simulink model "Speed_control_of_wound_field_synchronous_motor_drive"  (R2024a)
settings: Solver=FixedStepDiscrete  StartTime=0.0  StopTime=1  FixedStep=Ts  RelTol=1e-3  EnableMultiTasking=on
PreLoadFcn:
  | SMDriveData;
undefined symbols (not defined in the file): Kt, Ts
libraries: nesl_utility x15, fl_lib x10, ee_lib x6, eeSmFieldOrientedControl x1, batteryecm_lib x1
CloseFcn:
  | try,close(h1_SMDrive),end
  | clear h1_SMDrive
  | 
  | clear simlog_SMDrive
  | clear logsout_SMDrive
Description:
  | Three-Phase Synchronous Machine Drive
settings Model: Creator=The MathWorks, Inc.  LastModifiedBy=haris
settings SolverCC: AlgebraicLoopSolver=TrustRegion  AutoInsertRateTranBlk=on  MaxZcPerStep=1
settings DataIOCC: MaxDataPoints=210000  ReturnWorkspaceOutputs=off  SignalLoggingName=logsout_SMDrive
settings OptimizationCC: ReuseModelBlockBuffer=off  LifeSpan=inf
settings DebuggingCC: UnconnectedInputMsg=warning  UnconnectedOutputMsg=warning  UnconnectedLineMsg=warning  SFUnexpectedBacktrackingDiag=warning  SFNoUnconditionalDefaultTransitionDiag=warning  SFExecutionAtInitializationDiag=none  ArithmeticOperatorsInVariantConditions=warning
settings ModelReferenceCC: EnableRefExpFcnMdlSchedulingChecks=on
settings SFSimCC: SimUseLocalCustomCode=off  CustomCodeUndefinedFunction=UseInterfaceOnly
settings RTWCC: RTWUseLocalCustomCode=off  GPUComputeCapability=3.5  DLArmComputeVersion=19.05
settings CodeAppCC: StateflowObjectComments=on
settings GRTTargetCC: TargetLangStandard=C89/C90 (ANSI)
settings ConfigComp: CovMetricSettings=dw  CovSaveCumulativeToWorkspaceVar=on  CovSaveSingleToWorkspaceVar=on  CovExternalEMLEnable=off
settings SimscapeCC: SimscapeLogType=all  SimscapeLogSimulationStatistics=on  SimscapeLogName=simlog_SMDrive  SimscapeLogDataHistory=210000

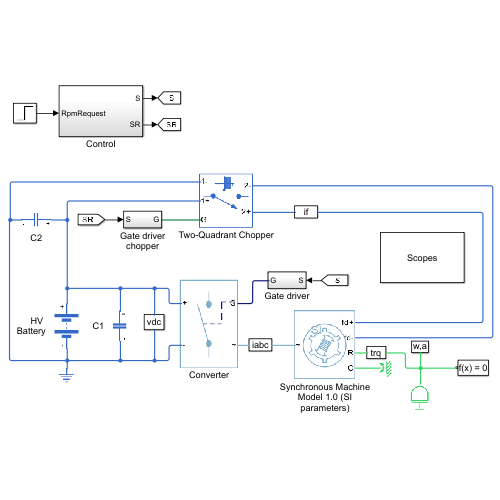
[thumbnail: Simulink's stored preview of the top-level diagram]
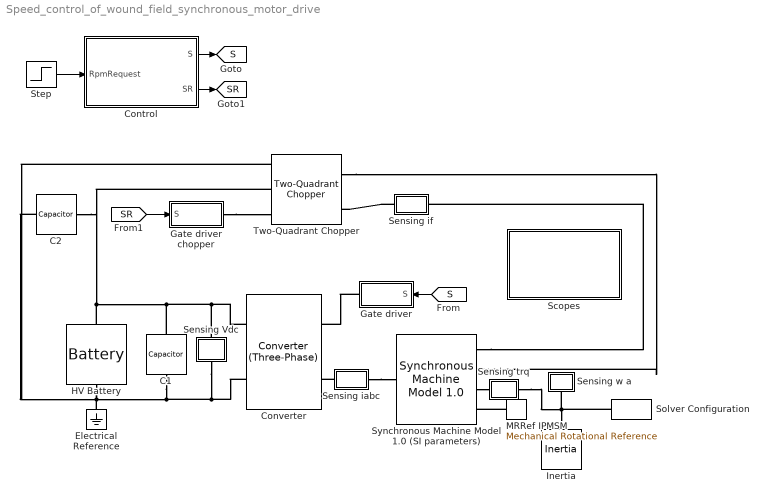
== system Speed_control_of_wound_field_synchronous_motor_drive ==
  C1 : fl_lib/Electrical/Electrical Elements/Capacitor  c=Cdc F  r=1e-6 Ohm  g=0 1/Ohm  i_specify=off  i_priority=None  i=0 A  i_nominal_specify=off  i_nominal_value=1  i_nominal_unit=A  v_specify=off  v_priority=None  v=0 V  v_nominal_specify=off  v_nominal_value=1  v_nominal_unit=V  vc_specify=on  vc_priority=None  vc=Vnom V  vc_nominal_specify=off  vc_nominal_value=1  vc_nominal_unit=V
  C2 : fl_lib/Electrical/Electrical Elements/Capacitor  c=Cdc F  r=1e-6 Ohm  g=0 1/Ohm  i_specify=off  i_priority=None  i=0 A  i_nominal_specify=off  i_nominal_value=1  i_nominal_unit=A  v_specify=off  v_priority=None  v=0 V  v_nominal_specify=off  v_nominal_value=1  v_nominal_unit=V  vc_specify=on  vc_priority=None  vc=Vnom V  vc_nominal_specify=off  vc_nominal_value=1  vc_nominal_unit=V
  Control : Subsystem
  Converter : ee_lib/Semiconductors & Converters/Converters/Converter (Three-Phase)  port_option=ee.enum.threePhasePort.composite  fidelity_option=ee.enum.converters.fidelity.detailed  device_type=2  K=0  Vf=0.8 V  Ron=0.001 Ohm  Rds=0.001 Ohm  Goff=1e-5 1/Ohm  Vgt=1 V  Vgt_off=-1 V  Ih=1 A  Vth=0.5 V  diode_param=2  diode_Vf=0.8 V  diode_Ron=0.001 Ohm  diode_Goff=1e-5 1/Ohm  diode_C=50 nF  diode_iRM=-235 A  diode_iF=300 A  diode_idot=-50 A/us  diode_trr_param=1  diode_trr_factor=3  diode_trr=15 us  diode_Qrr=1.5e+3 s*uA  snubber_type=0  Cs=1e-7 F  Rs=0.1 Ohm
  Electrical Reference : fl_lib/Electrical/Electrical Elements/Electrical Reference
  Gate driver : Subsystem
  Gate driver chopper : Subsystem
  HV Battery : batteryecm_lib/Battery  Vnom=Vnom V  prm_dir=1  R1_dis=2 Ohm  R1_ch=2 Ohm  R1=0.001 Ohm  prm_AH=1  AH=300 hr*A  V1=330 V  AH1=100 hr*A  prm_R2=1  R2=2000 Ohm  Tmeas=298.15 K  charge_measurement_port=simscape.enum.battery.enable.no  prm_dyn=1  Rp1=0.005 Ohm  tau1=30 s  Rp2=0.005 Ohm  tau2=30 s  Rp3=0.005 Ohm  tau3=30 s  Rp4=0.005 Ohm  tau4=30 s  Rp5=0.005 Ohm  tau5=30 s  prm_fade=1  N_fade=100  AH_fade=45 hr*A  R1_fade=2.02 Ohm  R1_ch_fade=2.02 Ohm  V1_fade=10.35 V  prm_age=1  prm_age_OCV=1  OCV_age=0.9  SOC_age=60  Tmeas_age=298.15 K  delta_time_age_vec=[0] d  temperature_age_vec=[273] K  OCV_scaling_age=2.2134e6  OCV_offset_age=1.632e6  temp_exp_age=0.515833569 V  t_exp_age=0.75  Vnom_T2=12 V  R1_T2=2.2 Ohm  R1_T2_dis=2.2 Ohm  R1_T2_ch=2.2 Ohm  V1_T2=11.4 V  R2_T2=2200 Ohm  Rp1_T2=0.005 Ohm  tau1_T2=30 s  Rp2_T2=0.005 Ohm  tau2_T2=30 s  Rp3_T2=0.005 Ohm  tau3_T2=30 s  Rp4_T2=0.005 Ohm  tau4_T2=30 s  Rp5_T2=0.005 Ohm  tau5_T2=30 s  Tmeas2=273.15 K  thermal_port=simscape.enum.thermaleffects.omit  thermal_mass=30000 J/K  i_specify=off  i_priority=None  i=0 A  i_nominal_specify=off  i_nominal_value=1  i_nominal_unit=A  v_specify=off  v_priority=None  v=0 V  v_nominal_specify=off  v_nominal_value=1  v_nominal_unit=V  charge_specify=on  charge_priority=High  charge=100 hr*A  charge_nominal_specify=off  charge_nominal_value=1  charge_nominal_unit=A*hr  num_cycles_specify=off  num_cycles_priority=High  num_cycles=0  num_cycles_nominal_specify=off  num_cycles_nominal_value=1  num_cycles_nominal_unit=1  temperature_specify=off  temperature_priority=High  temperature=298.15 K  temperature_nominal_specify=off  temperature_nominal_value=1  temperature_nominal_unit=K
  Inertia : fl_lib/Mechanical/Rotational Elements/Inertia  inertia=Jm kg*m^2  num_ports=foundation.enum.numPorts2.one  w_specify=on  w_priority=High  w=0 rpm  w_nominal_specify=off  w_nominal_value=1  w_nominal_unit=rad/s  t_specify=off  t_priority=High  t=0 N*m  t_nominal_specify=off  t_nominal_value=1  t_nominal_unit=N*m
  MRRef IPMSM : fl_lib/Mechanical/Rotational Elements/Mechanical Rotational Reference
  Scopes : Subsystem
      mask Display: disp(get_param(gcb,'Name'))
  Sensing Vdc : Subsystem
      mask Display: disp('vdc')
  Sensing trq : Subsystem
      mask Display: disp('trq')
  Sensing w a : Subsystem
      mask Display: disp('w,a')
  Sensing iabc : Subsystem
      mask Display: disp('iabc')
  Sensing if : Subsystem
      mask Display: disp('if')
  Solver Configuration : nesl_utility/Solver Configuration  PhysicalDomain=network_engine_domain  SubClassName=solver  LeftPortType=input  RightPortType=generic  Tones=[]  Harmonics=[]  SimulateNoise=off  Profile=off  UseLocalSampling=off  EnableSwitchedLinearOptims=on  FrequencyDomain=off  UseCCode=off  RelTol=0.001  AbsTol=1e-06  MinStep=1e-09  ToWorkspace=off  RevertToSquareIcSolve=off  NumHomotopyIterations=100  PhasorMode=off  PhasorModeNumHarmonics=1  ConsistencySolver=NEWTON_FTOL  IndexReductionMethod=DerivativeReplacement  DoDC=off  ResidualTolerance=1e-9  ConsistencyTolSource=GLOBAL  ConsistencyAbsTol=0.001  ConsistencyRelTol=0.001  ConsistencyTolFactor=0.001  UseLocalSolver=on  LocalSolverChoice=NE_BACKWARD_EULER_ADVANCER  ResolveIndetEquations=on  FunctionEvalNumThread=1  LocalSolverSampleTime=Ts  DoFixedCost=on  MaxNonlinIter=4  MaxModeIter=2  ComputeImpulses=off  ImpulseIterations=2  LinearAlgebra=auto  LinearAlgebraNumThread=0  EquationFormulation=NE_TIME_EF  DelaysMemoryBudget=1024  AutomaticFiltering=on  FilteringTimeConstant=0.001  PartitionStorageMethod=AS_NEEDED  PartitionMemoryBudget=1024  PartitionMethod=FAST  MultibodyUseLocalSolver=off  MultibodyLocalSolverChoice=ODE1  MultibodyLocalSolverSampleTime=0.001
  Step : Step  Time=0.1  After=1500  SampleTime=0
  Synchronous Machine Model 1.0 (SI parameters) : ee_lib/Electromechanical/Synchronous/Synchronous Machine Model 1.0  port_option=ee.enum.threePhasePort.composite  winding_type=ee.enum.electromech.statorconfiguration.wye  machine_param=ee.enum.pmsm.hybridparameterization.constant  nPolePairs=p  stator_param=1  Ld=Ld H  Lq=Lq H  idVec=[-200, 0, 200] A  iqVec=[-200, 0, 200] A  ifVec=[-20, 0, 20] A  LdMatrix=0.00015 * ones(3, 3, 3) H  LqMatrix=0.00021 * ones(3, 3, 3) H  LmfMatrix=0.007 * ones(3, 3, 3) H  LfVec=0.5 * ones(1, 3) H  L0=L0 H  Ls=0.00016 H  Lm=-0.00002 H  Ms=0.00002 H  Lf=Lf H  Lmf=Lmf H  Rs=Rs Ohm  Rf=Rf Ohm  zero_sequence=ee.enum.park.zerosequence.exclude  J=0 kg*m^2  lam=0 N*m/(rad/s)  axes_param=1  i_d_specify=off  i_d_priority=None  i_d=0 A  i_d_nominal_specify=off  i_d_nominal_value=1  i_d_nominal_unit=A  i_q_specify=off  i_q_priority=None  i_q=0 A  i_q_nominal_specify=off  i_q_nominal_value=1  i_q_nominal_unit=A  i_f_specify=off  i_f_priority=None  i_f=0 A  i_f_nominal_specify=off  i_f_nominal_value=1  i_f_nominal_unit=A  torque_specify=off  torque_priority=None  torque=0 N*m  torque_nominal_specify=off  torque_nominal_value=1  torque_nominal_unit=N*m  angular_velocity_specify=on  angular_velocity_priority=High  angular_velocity=0 rpm  angular_velocity_nominal_specify=off  angular_velocity_nominal_value=1  angular_velocity_nominal_unit=rpm  angular_position_diff_specify=on  angular_position_diff_priority=High  angular_position_diff=0 deg  angular_position_diff_nominal_specify=off  angular_position_diff_nominal_value=1  angular_position_diff_nominal_unit=deg  Tmeas=298.15 K  alpha=3.93e-3 1/K  stator_thermal_mass=100 J/K  rotor_thermal_mass=200 J/K  temperatureA_specify=off  temperatureA_priority=High  temperatureA=25 degC  temperatureA_nominal_specify=off  temperatureA_nominal_value=1  temperatureA_nominal_unit=degC  temperatureB_specify=off  temperatureB_priority=High  temperatureB=25 degC  temperatureB_nominal_specify=off  temperatureB_nominal_value=1  temperatureB_nominal_unit=degC  temperatureC_specify=off  temperatureC_priority=High  temperatureC=25 degC  temperatureC_nominal_specify=off  temperatureC_nominal_value=1  temperatureC_nominal_unit=degC  temperatureR_specify=off  temperatureR_priority=High  temperatureR=25 degC  temperatureR_nominal_specify=off  temperatureR_nominal_value=1  temperatureR_nominal_unit=degC
      settings: InternalSimscapePortConfiguration="{\"Bottom\":[],\"Left\":[{\"id\":\"N\",\"label\":\"~\",\"type\":\"foundation.electrical.three_phase\"}],\"Right\":[{\"id\":\"fd_p\",\"label\":\"fd+\",\"type\":\"foundation.electrical.electrical\"},{\"id\":\"fd_n\",\"label\":\"fd-\",\"type\":\"foundation.electrical.electrical\"},{\"id\":\"R\",\"label\":\"R\",\"type\":\"foundation.mechanical.rotational.rotational\"},{\"id\":\"C\",\"label\":\"C\",\"type\":\"foundation.mechanical.rotational.rotational\"}],\"Top\":[]}"
  Two-Quadrant Chopper : ee_lib/Semiconductors & Converters/Converters/Two-Quadrant Chopper  device_type=3  Vf=0.8 V  Ron=0.001 Ohm  Rds=0.001 Ohm  Goff=1e-5 1/Ohm  Vgt=1 V  Vgt_off=-1 V  Ih=1 A  Vth=0.5 V  K=0  diode_param=2  diode_Vf=0.8 V  diode_Ron=0.001 Ohm  diode_Goff=1e-5 1/Ohm  diode_C=50 nF  diode_iRM=-235 A  diode_iF=300 A  diode_idot=-50 A/us  diode_trr_param=1  diode_trr_factor=3  diode_trr=15 us  diode_Qrr=1500 s*uA  snubber_type=0  Cs=1e-7 F  Rs=0.1 Ohm
      settings: InternalSimscapePortConfiguration="{\"Bottom\":[],\"Left\":[{\"id\":\"G\",\"label\":\"G\",\"type\":\"foundation.electrical.four_phase\"},{\"id\":\"p1\",\"label\":\"1+\",\"type\":\"foundation.electrical.electrical\"},{\"id\":\"n1\",\"label\":\"1-\",\"type\":\"foundation.electrical.electrical\"}],\"Right\":[{\"id\":\"p2\",\"label\":\"2+\",\"type\":\"foundation.electrical.electrical\"},{\"id\":\"n2\",\"label\":\"2-\",\"type\":\"foundation.electrical.electrical\"}],\"Top\":[]}"
  tag scope: S=global, SR=global
  wires:
  [S] -> Gate driver/1(S)
  [SR] -> Gate driver chopper/1(S)
  Step/1 -> Control/1(RpmRequest)
  Control/1(S) -> [S]
  Control/2(SR) -> [SR]
  connections:
  Converter/RConn2 -- Sensing Vdc/RConn1 -- Two-Quadrant Chopper/LConn3 -- C2/RConn1 -- HV Battery/RConn1 -- Electrical Reference/LConn1 -- C1/RConn1
  Converter/RConn1 -- Sensing Vdc/LConn1 -- Two-Quadrant Chopper/LConn2 -- C2/LConn1 -- HV Battery/LConn1 -- C1/LConn1
  Gate driver/RConn1 -- Converter/LConn1
  Synchronous Machine Model 1.0 (SI parameters)/RConn1 -- Sensing if/RConn1
  Sensing iabc/LConn1 -- Converter/LConn2
  Sensing iabc/RConn1 -- Synchronous Machine Model 1.0 (SI parameters)/LConn1
  Solver Configuration/RConn1 -- Inertia/LConn1 -- Sensing trq/RConn1 -- Sensing w a/LConn1
  Synchronous Machine Model 1.0 (SI parameters)/RConn3 -- Sensing trq/LConn1
  MRRef IPMSM/LConn1 -- Synchronous Machine Model 1.0 (SI parameters)/RConn4
  Gate driver chopper/RConn1 -- Two-Quadrant Chopper/LConn1
  Two-Quadrant Chopper/RConn2 -- Synchronous Machine Model 1.0 (SI parameters)/RConn2
  Sensing if/LConn1 -- Two-Quadrant Chopper/RConn1

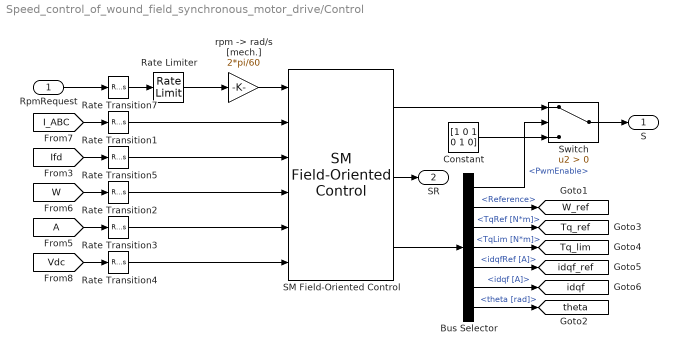
== system Speed_control_of_wound_field_synchronous_motor_drive/Control ==
  RpmRequest : Inport
  Bus Selector : BusSelector  OutputSignals=PwmEnable,Reference,TqRef [N*m],TqLim [N*m],idqfRef [A],idqf [A],theta [rad]
  Constant : Constant  Value=[1 0 1 0 1 0]
  From5 : From  TagVisibility=global
  Rate Limiter : RateLimiter  RisingSlewLimit=4000  FallingSlewLimit=-4000  SampleTimeMode=inherited
  Rate Transition{1..5,7} (6 alike) : RateTransition  OutPortSampleTime=Tsc
  SM Field-Oriented Control : eeSmFieldOrientedControl/SM Field-Oriented Control  CtrlMode=Velocity control  Vnom=Vnom  Pmax=Pmax  Tmax=Tmax  ifmax=ifmax  Vdc_on=100  p=p  Ts=Ts  Tsc=Tsc  CtrlType=PI control  Kp_w=Kp_omega  Ki_w=Ki_omega  Kv_w=1  Kaw_w=Kaw_omega  RefType=Zero d-axis control  rpmVec=[0, 3000]  TqVec=[-100, 0, 100]  VdcVec=[300, 350]  idMatrix=zeros(2,3,2)  iqMatrix=zeros(2,3,2)  ifMatrix=zeros(2,3,2)  Kt=Kt  AxisAlignment=Q-axis  Kp_id=Kp_id  Ki_id=Ki_id  Kaw_id=Kaw_id  Kp_iq=Kp_iq  Ki_iq=Ki_iq  Kaw_iq=Kaw_iq  Kp_if=Kp_if  Ki_if=Ki_if  Kaw_if=Kaw_if  AxisPrio=Q-axis  ActZC=on  ActFF=on  ParamTypeFF=Constant parameters  Ld=Ld  Lq=Lq  Lmf=Lmf  idVect=[-200, 200]  iqVect=[-200, 200]  ifVect=[0, 20]  LdMatrix=0.0002 * ones(2,2,2)  LqMatrix=0.0002 * ones(2,2,2)  LmfMatrix=0.007 * ones(2,2,2)  CPWMMode=SVM: space vector modulation  fsw=fsw  ChopperType=First and fourth quadrant chopper  fswe=fsw
      settings: SamplingMode=Natural
  Switch : Switch  Criteria=u2 > Threshold  SaturateOnIntegerOverflow=off  InputSameDT=off
  "rpm -> rad/s [mech.]" : Gain  Gain=2*pi/60
  S : Outport  VectorParamsAs1DForOutWhenUnconnected=off
  SR : Outport  Port=2  VectorParamsAs1DForOutWhenUnconnected=off
  tag scope: Tq_lim=global, Tq_ref=global, W_ref=global, idqf=global, idqf_ref=global, theta=global
  wires:
  [Ifd] -> Rate Transition5/1
  [W] -> Rate Transition2/1
  Rate Transition1/1 -> SM Field-Oriented Control/2
  [I_ABC] -> Rate Transition1/1
  From5/1 -> Rate Transition3/1
  RpmRequest/1 -> Rate Transition7/1
  [Vdc] -> Rate Transition4/1
  Rate Transition7/1 -> Rate Limiter/1
  "rpm -> rad/s [mech.]"/1 -> SM Field-Oriented Control/1
  SM Field-Oriented Control/2 -> SR/1
  SM Field-Oriented Control/3 -> Bus Selector/1
  Bus Selector/2 -> [W_ref]  "<Reference>"
  Bus Selector/7 -> [theta]  "<theta [rad]>"
  Bus Selector/3 -> [Tq_ref]  "<TqRef [N*m]>"
  Bus Selector/4 -> [Tq_lim]  "<TqLim [N*m]>"
  Bus Selector/5 -> [idqf_ref]  "<idqfRef [A]>"
  Bus Selector/6 -> [idqf]  "<idqf [A]>"
  Rate Limiter/1 -> "rpm -> rad/s [mech.]"/1
  Rate Transition5/1 -> SM Field-Oriented Control/3
  Rate Transition2/1 -> SM Field-Oriented Control/4
  Rate Transition3/1 -> SM Field-Oriented Control/5
  Rate Transition4/1 -> SM Field-Oriented Control/6
  SM Field-Oriented Control/1 -> Switch/1
  Switch/1 -> S/1
  Constant/1 -> Switch/3
  Bus Selector/1 -> Switch/2  "<PwmEnable>"

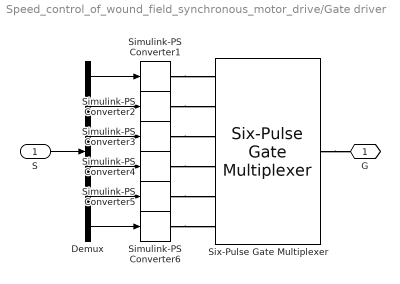
== system Speed_control_of_wound_field_synchronous_motor_drive/Gate driver ==
  S : Inport
  Demux : Demux  Outputs=6
  Simulink-PS Converter{1..6} (6 alike) : nesl_utility/Simulink-PS Converter  PhysicalDomain=network_engine_domain  SubClassName=ps_input  LeftPortType=input  RightPortType=output  PseudoPeriodic=off  Frequencies=[]  NoiseDistribution=none  NoiseParameters=[]  Unit=1  AffineConversion=off  FilteringAndDerivatives=zero  SimscapeFilterOrder=1  InputFilterTimeConstant=0.001  UdotUserProvided=1
  Six-Pulse Gate Multiplexer : ee_lib/Semiconductors & Converters/Converters/Six-Pulse Gate Multiplexer  port_option=ee.enum.controlport.ps
  G : PMIOPort  Side=Right
  wires:
  Demux/1 -> Simulink-PS Converter1/1
  S/1 -> Demux/1
  Demux/4 -> Simulink-PS Converter4/1
  Demux/2 -> Simulink-PS Converter2/1
  Demux/3 -> Simulink-PS Converter3/1
  Demux/5 -> Simulink-PS Converter5/1
  Demux/6 -> Simulink-PS Converter6/1
  connections:
  Six-Pulse Gate Multiplexer/RConn1 -- G/RConn1
  Simulink-PS Converter1/RConn1 -- Six-Pulse Gate Multiplexer/LConn1
  Simulink-PS Converter3/RConn1 -- Six-Pulse Gate Multiplexer/LConn3
  Simulink-PS Converter5/RConn1 -- Six-Pulse Gate Multiplexer/LConn5
  Simulink-PS Converter6/RConn1 -- Six-Pulse Gate Multiplexer/LConn6
  Simulink-PS Converter4/RConn1 -- Six-Pulse Gate Multiplexer/LConn4
  Simulink-PS Converter2/RConn1 -- Six-Pulse Gate Multiplexer/LConn2

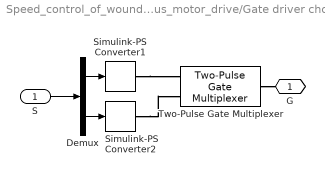
== system Speed_control_of_wound_field_synchronous_motor_drive/Gate driver chopper ==
  S : Inport
  Demux : Demux  Outputs=2
  Simulink-PS Converter1 : nesl_utility/Simulink-PS Converter  PhysicalDomain=network_engine_domain  SubClassName=ps_input  LeftPortType=input  RightPortType=output  PseudoPeriodic=off  Frequencies=[]  NoiseDistribution=none  NoiseParameters=[]  Unit=1  AffineConversion=off  FilteringAndDerivatives=zero  SimscapeFilterOrder=1  InputFilterTimeConstant=0.001  UdotUserProvided=1
  Simulink-PS Converter2 : nesl_utility/Simulink-PS Converter  PhysicalDomain=network_engine_domain  SubClassName=ps_input  LeftPortType=input  RightPortType=output  PseudoPeriodic=off  Frequencies=[]  NoiseDistribution=none  NoiseParameters=[]  Unit=1  AffineConversion=off  FilteringAndDerivatives=zero  SimscapeFilterOrder=1  InputFilterTimeConstant=0.001  UdotUserProvided=1
  Two-Pulse Gate Multiplexer : ee_lib/Semiconductors & Converters/Converters/Two-Pulse Gate Multiplexer  port_option=ee.enum.controlport.ps
      settings: InternalSimscapePortConfiguration="{\"Bottom\":[],\"Left\":[{\"id\":\"G1_ps\",\"label\":\"G1\",\"type\":\"input\"},{\"id\":\"G2_ps\",\"label\":\"G2\",\"type\":\"input\"}],\"Right\":[{\"id\":\"p\",\"label\":\"G\",\"type\":\"foundation.electrical.four_phase\"}],\"Top\":[]}"
  G : PMIOPort  Side=Right
  wires:
  Demux/1 -> Simulink-PS Converter1/1
  Demux/2 -> Simulink-PS Converter2/1
  S/1 -> Demux/1
  connections:
  Two-Pulse Gate Multiplexer/RConn1 -- G/RConn1
  Simulink-PS Converter1/RConn1 -- Two-Pulse Gate Multiplexer/LConn1
  Simulink-PS Converter2/RConn1 -- Two-Pulse Gate Multiplexer/LConn2

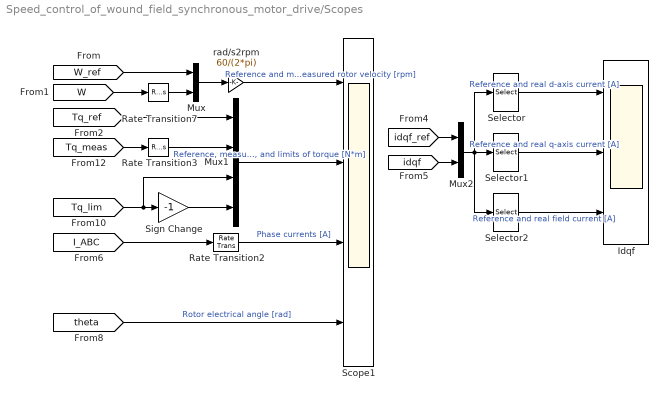
== system Speed_control_of_wound_field_synchronous_motor_drive/Scopes ==
  "Idqf " : Scope  NumInputPorts=3
  Mux : Mux  Inputs=2
  Mux1 : Mux
  Mux2 : Mux  Inputs=2
  Rate Transition2 : RateTransition
  Rate Transition3 : RateTransition
  Rate Transition7 : RateTransition
  Scope1 : Scope  NumInputPorts=4
  Selector : Selector  InputPortWidth=6  IndexOptions=Index vector (dialog)  Indices=[1 4]  OutputSizes=1
  Selector1 : Selector  InputPortWidth=6  IndexOptions=Index vector (dialog)  Indices=[2 5]  OutputSizes=1
  Selector2 : Selector  InputPortWidth=6  IndexOptions=Index vector (dialog)  Indices=[3 6]  OutputSizes=1
  Sign Change : Gain  Gain=-1
  rad/s2rpm : Gain  Gain=60/(2*pi)
  wires:
  Mux1/1 -> Scope1/2  "Reference, measured, and limits of torque [N*m]"
  Sign Change/1 -> Mux1/4
  Rate Transition3/1 -> Mux1/2
  [idqf] -> Mux2/2
  [W] -> Rate Transition7/1
  Selector/1 -> "Idqf "/1  "Reference and real d-axis current [A]"
  [I_ABC] -> Rate Transition2/1
  [idqf_ref] -> Mux2/1
  [theta] -> Scope1/4  "Rotor electrical angle [rad]"
  Mux2/1 -> Selector/1, Selector2/1, Selector1/1
  Selector1/1 -> "Idqf "/2  "Reference and real q-axis current [A]"
  [W_ref] -> Mux/1
  [Tq_meas] -> Rate Transition3/1
  Selector2/1 -> "Idqf "/3  "Reference and real field current [A]"
  [Tq_lim] -> Mux1/3, Sign Change/1
  Mux/1 -> rad/s2rpm/1
  Rate Transition2/1 -> Scope1/3  "Phase currents [A]"
  [Tq_ref] -> Mux1/1
  rad/s2rpm/1 -> Scope1/1  "Reference and measured rotor velocity [rpm]"
  Rate Transition7/1 -> Mux/2

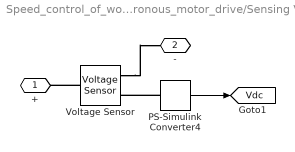
== system Speed_control_of_wound_field_synchronous_motor_drive/Sensing Vdc ==
  PS-Simulink Converter4 : nesl_utility/PS-Simulink Converter  PhysicalDomain=network_engine_domain  SubClassName=ps_output  LeftPortType=input  RightPortType=output  PseudoPeriodic=off  Frequencies=[]  VectorFormat=1-D array  Unit=V  AffineConversion=off
  Voltage Sensor : fl_lib/Electrical/Electrical Sensors/Voltage Sensor
  + : PMIOPort  Side=Left
  - : PMIOPort  Port=2  Side=Right
  tag scope: Vdc=global
  wires:
  PS-Simulink Converter4/1 -> [Vdc]
  connections:
  Voltage Sensor/LConn1 -- +/RConn1
  Voltage Sensor/RConn2 -- -/RConn1
  PS-Simulink Converter4/LConn1 -- Voltage Sensor/RConn1

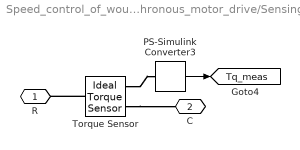
== system Speed_control_of_wound_field_synchronous_motor_drive/Sensing trq ==
  PS-Simulink Converter3 : nesl_utility/PS-Simulink Converter  PhysicalDomain=network_engine_domain  SubClassName=ps_output  LeftPortType=input  RightPortType=output  PseudoPeriodic=off  Frequencies=[]  VectorFormat=1-D array  Unit=N*m  AffineConversion=off
  Torque Sensor : fl_lib/Mechanical/Mechanical Sensors/Ideal Torque Sensor
  R : PMIOPort  Side=Left
  C : PMIOPort  Port=2  Side=Right
  tag scope: Tq_meas=global
  wires:
  PS-Simulink Converter3/1 -> [Tq_meas]
  connections:
  Torque Sensor/RConn1 -- C/RConn1
  Torque Sensor/RConn2 -- PS-Simulink Converter3/LConn1
  Torque Sensor/LConn1 -- R/RConn1

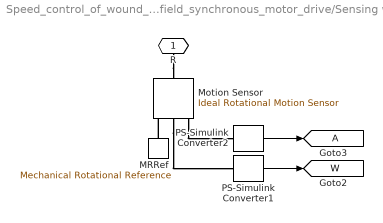
== system Speed_control_of_wound_field_synchronous_motor_drive/Sensing w a ==
  Goto3 : Goto  TagVisibility=global
  MRRef : fl_lib/Mechanical/Rotational Elements/Mechanical Rotational Reference
  Motion Sensor : fl_lib/Mechanical/Mechanical Sensors/Ideal Rotational Motion Sensor  reference=foundation.enum.MeasurementReference.difference  acceleration_port=false  velocity_port=true  position_port=true  wrap_angle=simscape.enum.onoff.off  offset=0 deg
  PS-Simulink Converter1 : nesl_utility/PS-Simulink Converter  PhysicalDomain=network_engine_domain  SubClassName=ps_output  LeftPortType=input  RightPortType=output  PseudoPeriodic=off  Frequencies=[]  VectorFormat=1-D array  Unit=rad/s  AffineConversion=off
  PS-Simulink Converter2 : nesl_utility/PS-Simulink Converter  PhysicalDomain=network_engine_domain  SubClassName=ps_output  LeftPortType=input  RightPortType=output  PseudoPeriodic=off  Frequencies=[]  VectorFormat=1-D array  Unit=rad  AffineConversion=off
  R : PMIOPort  Side=Left
  tag scope: W=global
  wires:
  PS-Simulink Converter1/1 -> [W]
  PS-Simulink Converter2/1 -> Goto3/1
  connections:
  R/RConn1 -- Motion Sensor/LConn1
  Motion Sensor/RConn2 -- PS-Simulink Converter1/LConn1
  MRRef/LConn1 -- Motion Sensor/RConn1
  Motion Sensor/RConn3 -- PS-Simulink Converter2/LConn1

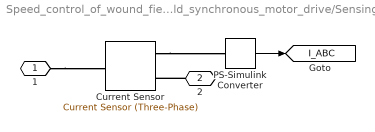
== system Speed_control_of_wound_field_synchronous_motor_drive/Sensing iabc ==
  Current Sensor : ee_lib/Sensors & Transducers/Current Sensor (Three-Phase)
  PS-Simulink Converter : nesl_utility/PS-Simulink Converter  PhysicalDomain=network_engine_domain  SubClassName=ps_output  LeftPortType=input  RightPortType=output  PseudoPeriodic=off  Frequencies=[]  VectorFormat=1-D array  Unit=A  AffineConversion=off
  1 : PMIOPort  Side=Left
  2 : PMIOPort  Port=2  Side=Right
  tag scope: I_ABC=global
  wires:
  PS-Simulink Converter/1 -> [I_ABC]
  connections:
  1/RConn1 -- Current Sensor/LConn1
  2/RConn1 -- Current Sensor/RConn2
  Current Sensor/RConn1 -- PS-Simulink Converter/LConn1

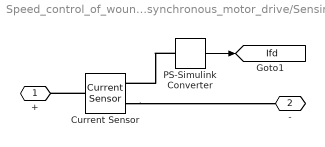
== system Speed_control_of_wound_field_synchronous_motor_drive/Sensing if ==
  Current Sensor : fl_lib/Electrical/Electrical Sensors/Current Sensor
  PS-Simulink Converter : nesl_utility/PS-Simulink Converter  PhysicalDomain=network_engine_domain  SubClassName=ps_output  LeftPortType=input  RightPortType=output  PseudoPeriodic=off  Frequencies=[]  VectorFormat=1-D array  Unit=1  AffineConversion=off
  + : PMIOPort  Side=Left
  - : PMIOPort  Port=2  Side=Right
  tag scope: Ifd=global
  wires:
  PS-Simulink Converter/1 -> [Ifd]
  connections:
  Current Sensor/LConn1 -- +/RConn1
  Current Sensor/RConn2 -- -/RConn1
  PS-Simulink Converter/LConn1 -- Current Sensor/RConn1
